simulink model "si_pneumatic_physical"  (R2025b)
settings: Solver=ode45  StartTime=0.0  StopTime=2  MaxStep=.005  RelTol=1e-9  AbsTol=1e-11
model workspace (MAT data in the model file):
  p.area = 0.0028
  p.half_stroke = 0.125
  p.midpoint_volume = 0.0005
  p.piston_mass = 2.9
  p.load_mass = 3
  p.viscous = 135
  p.coulomb = 21
  p.valve_gain = 0.0001
  p.voltage_limit = 10
  p.supply_pressure = 900000
  p.exhaust_pressure = 100000
  p.reservoir_temperature = 293.15
  p.universal_R = 8.31446261815
  p.air_molar_mass = 0.0289644
  p.gamma = 1.4
  p.gravity = 9.81
  p.port_width = 0.002
  p.discharge_coefficient = 0.7
  p.bypass_area = 0
  p.friction_velocity = 0.005
  p.wall_conductance = 0
  p.wall_temperature = 293.15
  xinit = [0; 0; 0.00303225881629; 0.00290943758556; 293.15; 293.15]
settings Model: Creator=runner  LastModifiedBy=runner
settings DataIOCC: OutputOption=SpecifiedOutputTimes  OutputTimes=0:.01:2

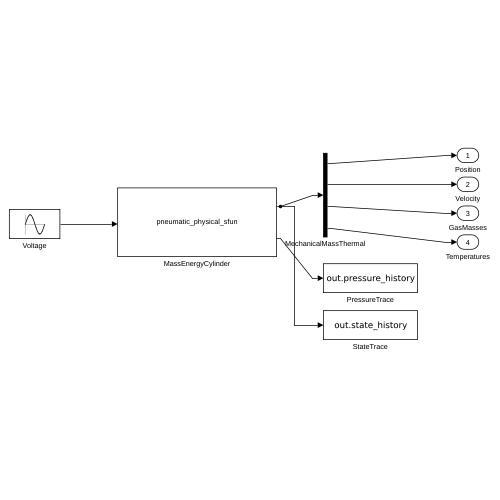
[thumbnail: Simulink's stored preview of the top-level diagram]
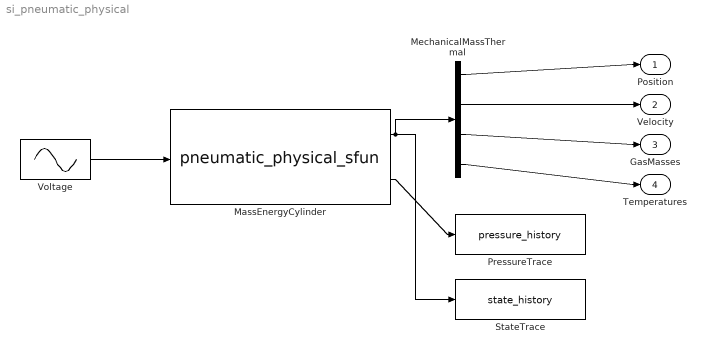
== system si_pneumatic_physical ==
  MassEnergyCylinder : M-S-Function  FunctionName=pneumatic_physical_sfun  Parameters=xinit,p
  MechanicalMassThermal : Demux  Outputs=[1 1 2 2]
  PressureTrace : ToWorkspace  VariableName=pressure_history  SaveFormat=Structure With Time  SampleTime=-1
  StateTrace : ToWorkspace  VariableName=state_history  SaveFormat=Structure With Time  SampleTime=-1
  Voltage : Sin  Amplitude=2  Frequency=2*pi  SampleTime=0
  Position : Outport
  Velocity : Outport  Port=2
  GasMasses : Outport  Port=3
  Temperatures : Outport  Port=4
  wires:
  MechanicalMassThermal/1 -> Position/1
  MechanicalMassThermal/2 -> Velocity/1
  MechanicalMassThermal/3 -> GasMasses/1
  MechanicalMassThermal/4 -> Temperatures/1
  Voltage/1 -> MassEnergyCylinder/1
  MassEnergyCylinder/1 -> MechanicalMassThermal/1, StateTrace/1
  MassEnergyCylinder/2 -> PressureTrace/1
